simulink model "qnet_hvac_simulink"  (R2026a)
settings: Solver=ode45  StopTime=360.0  RelTol=1e-4  AbsTol=1e-6
libraries: slpidlib x1
settings Model: Creator=Fufal Jigar  LastModifiedBy=Fufal Jigar

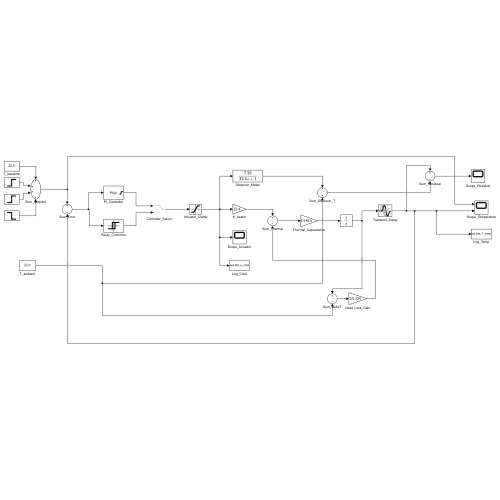
[thumbnail: Simulink's stored preview of the top-level diagram]
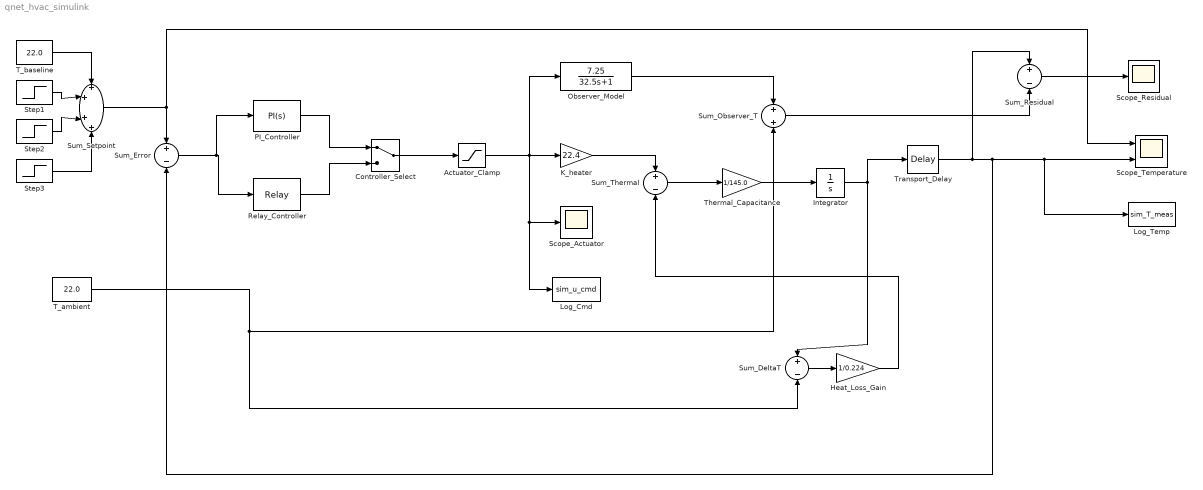
== system qnet_hvac_simulink ==
  Actuator_Clamp : Saturate  UpperLimit=5.0  LowerLimit=0.0
  Controller_Select : ManualSwitch
  Heat_Loss_Gain : Gain  Gain=1/0.224
  Integrator : Integrator  InitialCondition=22.0
  K_heater : Gain  Gain=22.4
  Log_Cmd : ToWorkspace  VariableName=sim_u_cmd  SaveFormat=Timeseries  SampleTime=-1
  Log_Temp : ToWorkspace  VariableName=sim_T_meas  SaveFormat=Timeseries  SampleTime=-1
  Observer_Model : TransferFcn  Numerator=[7.25]  Denominator=[32.5 1]
  PI_Controller : slpidlib/PID Controller  Controller=PI  Form=Parallel  TimeDomain=Continuous-time  UseExternalTs=off  SampleTime=-1  IntegratorMethod=Forward Euler  FilterMethod=Forward Euler  ControllerParametersSource=internal  P=1.35  I=0.042  UseKiTs=off  D=0  UseExternalDerivativeSource=off  N=100  UseFilter=on  TunerSelectOption=Transfer Function Based (PID Tuner App)  InitialConditionSource=internal  InitialConditionForIntegrator=0  InitialConditionForFilter=0  DifferentiatorICPrevScaledInput=0  ExternalReset=none  TrackingMode=off  Kt=1  LimitOutput=on  SatLimitsSource=internal  UpperSaturationLimit=5.0  LowerSaturationLimit=0.0  LinearizeAsGain=on  AntiWindupMode=clamping  Kb=1  LimitIntegrator=off  UpperIntegratorSaturationLimit=inf  LowerIntegratorSaturationLimit=-inf  POutMin=[]  POutMax=[]  IOutMin=[]  IOutMax=[]  DOutMin=[]  DOutMax=[]  NOutMin=[]  NOutMax=[]  SumOutMin=[]  SumOutMax=[]  SaturationOutMin=[]  SaturationOutMax=[]  PParamMin=[]  PParamMax=[]  IParamMin=[]  IParamMax=[]  DParamMin=[]  DParamMax=[]  NParamMin=[]  NParamMax=[]  KbParamMin=[]  KbParamMax=[]  KtParamMin=[]  KtParamMax=[]  KbOutMin=[]  KbOutMax=[]  KtOutMin=[]  KtOutMax=[]  IntegratorOutMin=[]  IntegratorOutMax=[]  FilterOutMin=[]  FilterOutMax=[]  SumI1OutMin=[]  SumI1OutMax=[]  SumI2OutMin=[]  SumI2OutMax=[]  SumI3OutMin=[]  SumI3OutMax=[]  SumI4OutMin=[]  SumI4OutMax=[]  SumDOutMin=[]  SumDOutMax=[]  DifferentiatorOutMin=[]  DifferentiatorOutMax=[]  FilterDiffOutCoefMin=[]  FilterDiffOutCoefMax=[]  ReciprocalOutMin=[]  ReciprocalOutMax=[]  SumDenOutMin=[]  SumDenOutMax=[]  SumNumOutMin=[]  SumNumOutMax=[]  DivideOutMin=[]  DivideOutMax=[]  UdiffTsProdOutMin=[]  UdiffTsProdOutMax=[]  NTsProdOutMin=[]  NTsProdOutMax=[]  UintegralTsProdOutMin=[]  UintegralTsProdOutMax=[]  UngainTsProdOutMin=[]  UngainTsProdOutMax=[]  ClampingZeroOutDataTypeStr=Inherit: Inherit via back propagation  ClampingZeroOutMin=[]  ClampingZeroOutMax=[]  FilterDenConstantOutDataTypeStr=Inherit: Inherit via back propagation  FilterDenConstantOutMin=[]  FilterDenConstantOutMax=[]  PCopyOutDataTypeStr=Inherit: Inherit via back propagation  PCopyOutMin=[]  PCopyOutMax=[]  NCopyOutDataTypeStr=Inherit: Inherit via back propagation  NCopyOutMin=[]  NCopyOutMax=[]  IntegratorContinuousStateAttributes=''  IntegratorStateMustResolveToSignalObject=off  IntegratorRTWStateStorageClass=Auto  FilterContinuousStateAttributes=''  FilterStateMustResolveToSignalObject=off  FilterRTWStateStorageClass=Auto  ParallelPVariant=InternalParameters  IdealPVariant=Disabled  IVariant=InternalParameters  DVariant=Disabled  IntegratorVariant=Continuous  SatVariant=Enabled  AWVariant=ContClampingParallel  PCopyVariant=Disabled  TRVariant=Disabled  FdbkBlocksVariant=Forward  IdealPFdbkVariant=Disabled  SatFdbkVariant=Disabled  DerivativeFilterVariant=Disabled  NVariant=Disabled  NCopyVariant=Disabled_SignalSpec  FilterICVariant=Disabled  IntegratorICVariant=InternalICs  ExternalResetVariant=Disabled  TRSumVariant=Passthrough  SumFdbkVariant=Disabled  SumVariant=Sum_PI  TsampFilterVariant=InternalTs  TsampNgainVariant=Passthrough  TsampIntegralVariant=Disabled_SignalSpec  ExternalSaturationOutDataTypeStr=Inherit: Same as second input  DerivativeSourceVariant=Disabled  PreIntVariant=InternalPreInt
  Relay_Controller : Relay  OnSwitchValue=0.4  OffSwitchValue=-0.4  OnOutputValue=5.0  OffOutputValue=0.0
  Scope_Actuator : Scope
  Scope_Residual : Scope
  Scope_Temperature : Scope  NumInputPorts=2
  Step1 : Step  Time=20.0  InitialValue=0.0  FinalValue=10.0  SampleTime=0
  Step2 : Step  Time=140.0  InitialValue=0.0  FinalValue=10.0  SampleTime=0
  Step3 : Step  Time=260.0  InitialValue=0.0  FinalValue=-6.0  SampleTime=0
  Sum_DeltaT : Sum  Inputs=+-
  Sum_Error : Sum  Inputs=+-
  Sum_Observer_T : Sum
  Sum_Residual : Sum  Inputs=+-
  Sum_Setpoint : Sum  Inputs=++++
  Sum_Thermal : Sum  Inputs=+-
  T_ambient : Constant  Value=22.0
  T_baseline : Constant  Value=22.0
  Thermal_Capacitance : Gain  Gain=1/145.0
  Transport_Delay : TransportDelay  DelayTime=2.0  InitialOutput=22.0
  wires:
  T_baseline/1 -> Sum_Setpoint/1
  Step1/1 -> Sum_Setpoint/2
  Step2/1 -> Sum_Setpoint/3
  Step3/1 -> Sum_Setpoint/4
  Sum_Setpoint/1 -> Scope_Temperature/1, Sum_Error/1
  Sum_Error/1 -> Relay_Controller/1, PI_Controller/1
  PI_Controller/1 -> Controller_Select/1
  Relay_Controller/1 -> Controller_Select/2
  Controller_Select/1 -> Actuator_Clamp/1
  Actuator_Clamp/1 -> Log_Cmd/1, Scope_Actuator/1, K_heater/1, Observer_Model/1
  Observer_Model/1 -> Sum_Observer_T/1
  T_ambient/1 -> Sum_Observer_T/2, Sum_DeltaT/2
  Sum_Observer_T/1 -> Sum_Residual/2
  K_heater/1 -> Sum_Thermal/1
  Sum_Thermal/1 -> Thermal_Capacitance/1
  Thermal_Capacitance/1 -> Integrator/1
  Integrator/1 -> Sum_DeltaT/1, Transport_Delay/1
  Transport_Delay/1 -> Log_Temp/1, Scope_Temperature/2, Sum_Error/2, Sum_Residual/1
  Sum_Residual/1 -> Scope_Residual/1
  Sum_DeltaT/1 -> Heat_Loss_Gain/1
  Heat_Loss_Gain/1 -> Sum_Thermal/2
